simulink model "snap_adc5g_spec_rpi"  (R2019a)
settings: Solver=VariableStepDiscrete  StartTime=0.0  StopTime=10.0  RelTol=1e-3
undefined symbols (not defined in the file): pfb_coeff_gen_calc
libraries: xbsIndex_r4 x13965, casper_library_misc x80, casper_library_delays x43, xps_library x5, xbsReplacements_r4 x2, casper_library_communications x1
(part 94 of 152)

== system snap_adc5g_spec_rpi/fft_wideband_real/fft_direct/butterfly1_1/twiddle/coeff_gen/cosin ==
  theta : Inport
  misci : Inport  Port=2
  Constant : xbsIndex_r4/Constant  const=0  gui_display_data_type=Fixed-point  arith_type=Signed (2's comp)  n_bits=n_bits  bin_pt=bin_pt  preci_type=Single  exp_width=8  frac_width=24  explicit_period=off  period=1  equ=P=C  opselect=C  inp2=PCIN>>17  opr=+  inp1=P  carry=CIN  dbl_ovrd=off  block_type=constant
  Constant1 : xbsIndex_r4/Constant  const=0  gui_display_data_type=Fixed-point  arith_type=Signed (2's comp)  n_bits=n_bits  bin_pt=bin_pt  preci_type=Single  exp_width=8  frac_width=24  explicit_period=off  period=1  equ=P=C  opselect=C  inp2=PCIN>>17  opr=+  inp1=P  carry=CIN  dbl_ovrd=off  block_type=constant
  Constant2 : xbsIndex_r4/Constant  const=0  gui_display_data_type=Fixed-point  arith_type=Boolean  n_bits=n_bits  bin_pt=bin_pt  preci_type=Single  exp_width=8  frac_width=24  explicit_period=off  period=1  equ=P=C  opselect=C  inp2=PCIN>>17  opr=+  inp1=P  carry=CIN  dbl_ovrd=off  block_type=constant
  Constant3 : xbsIndex_r4/Constant  const=0  gui_display_data_type=Fixed-point  arith_type=Boolean  n_bits=n_bits  bin_pt=bin_pt  preci_type=Single  exp_width=8  frac_width=24  explicit_period=off  period=1  equ=P=C  opselect=C  inp2=PCIN>>17  opr=+  inp1=P  carry=CIN  dbl_ovrd=off  block_type=constant
  Constant4 : xbsIndex_r4/Constant  const=0  gui_display_data_type=Fixed-point  arith_type=Unsigned  n_bits=1  bin_pt=0  preci_type=Single  exp_width=8  frac_width=24  explicit_period=on  period=1  equ=P=C  opselect=C  inp2=PCIN>>17  opr=+  inp1=P  carry=CIN  dbl_ovrd=off  block_type=constant
  Constant5 : xbsIndex_r4/Constant  const=0  gui_display_data_type=Fixed-point  arith_type=Unsigned  n_bits=1  bin_pt=0  preci_type=Single  exp_width=8  frac_width=24  explicit_period=on  period=1  equ=P=C  opselect=C  inp2=PCIN>>17  opr=+  inp1=P  carry=CIN  dbl_ovrd=off  block_type=constant
  Delay : xbsIndex_r4/Delay  rst=off  infoeditControl=Selection of Reset will increase slice count due to use of real FFs and instead of SRLs  en=off  latency=bram_latency  reg_retiming=on  dbl_ovrd=off  block_type=delay
  Delay10 : xbsIndex_r4/Delay  rst=off  infoeditControl=Selection of Reset will increase slice count due to use of real FFs and instead of SRLs  en=off  latency=bram_latency  reg_retiming=on  dbl_ovrd=off  block_type=delay
  Delay8 : xbsIndex_r4/Delay  rst=off  infoeditControl=Selection of Reset will increase slice count due to use of real FFs and instead of SRLs  en=off  latency=bram_latency  reg_retiming=on  dbl_ovrd=off  block_type=delay
  Terminator : Terminator
  Terminator1 : Terminator
  add_convert0 : Subsystem
  add_convert1 : Subsystem
  assert : xbsIndex_r4/Assert  assert_type=on  type_source=Explicitly  gui_display_data_type=Fixed-point  arith_type=Unsigned  n_bits=11  bin_pt=0  preci_type=Single  exp_width=8  frac_width=24  assert_rate=off  rate_source=Explicitly  period=1  output_port=on  block_type=assert
  invert0 : Subsystem  mask{n_bits=n_bits, bin_pt=bin_pt, neg_latency=neg_latency, mux_latency=mux_latency}
      mask prompts: n_bits "bit width"; bin_pt "binary point"; neg_latency "negate latency"; mux_latency "mux latency"
  invert1 : Subsystem  mask{n_bits=n_bits, bin_pt=bin_pt, neg_latency=neg_latency, mux_latency=mux_latency}
      mask prompts: n_bits "bit width"; bin_pt "binary point"; neg_latency "negate latency"; mux_latency "mux latency"
  lookup : xbsIndex_r4/Dual Port RAM  depth=2^(11)  initVector=sin((0*(2*pi))+(2*pi)/(2^13)*(0:(2^11)-1))  distributed_mem=Block RAM  init_a=0  init_b=0  rst_a=off  rst_b=off  en_a=off  en_b=off  latency=bram_latency  write_mode_A=Read After Write  write_mode_B=Read After Write  optimize=Area  dbl_ovrd=off  block_type=dpram
  -sin : Outport
  -cos : Outport  Port=2
  misco : Outport  Port=3
  wires:
  theta/1 -> assert/1
  assert/1 -> add_convert0/1(theta), add_convert1/1(theta)
  Constant4/1 -> add_convert0/2(misci)
  add_convert0/3(misco) -> Terminator/1
  misci/1 -> add_convert1/2(misci)
  add_convert1/3(misco) -> Delay/1
  add_convert0/2(add) -> lookup/1
  add_convert1/2(add) -> lookup/4
  Constant/1 -> lookup/2
  Constant2/1 -> lookup/3
  Constant1/1 -> lookup/5
  Constant3/1 -> lookup/6
  add_convert1/1(negate) -> Delay8/1
  add_convert0/1(negate) -> Delay10/1
  Delay10/1 -> invert0/1(negate)
  Constant5/1 -> invert0/3(misci)
  lookup/1 -> invert0/2(in)
  Delay8/1 -> invert1/1(negate)
  lookup/2 -> invert1/2(in)
  invert0/2(misco) -> Terminator1/1
  Delay/1 -> invert1/3(misci)
  invert0/1(out) -> -sin/1
  invert1/1(out) -> -cos/1
  invert1/2(misco) -> misco/1

== system snap_adc5g_spec_rpi/fft_wideband_real/fft_unscrambler/reorder/buf0/rep_addr/bussify ==
  in1 : Inport
  in2 : Inport  Port=2
  in3 : Inport  Port=3
  in4 : Inport  Port=4
  in5 : Inport  Port=5
  in6 : Inport  Port=6
  in7 : Inport  Port=7
  in8 : Inport  Port=8
  concatenate : xbsIndex_r4/Concat  num_inputs=8  dbl_ovrd=off  block_type=concat
  reinterpret{1..8} (8 alike) : xbsIndex_r4/Reinterpret  force_arith_type=on  arith_type=Unsigned  force_bin_pt=on  bin_pt=0  block_type=reinterpret
      reinterpret1 settings: infoedit="Changes signal type without altering the binary representation.   You can changed the signal between signed and unsigned, and relocate the binary point.<br><br>Hardware notes: In hardware this block costs nothing.<br><br>Example:  Suppose the input is 6 bits wide, signed, with 2 fractional bits, and the output is forced to unsigned with 0 fractional bits.  Then an input of -2.0 (1110.00 in binary 2's complement) becomes an output of 56 (111000 in binary)."
      reinterpret2 settings: infoedit="Changes signal type without altering the binary representation.   You can changed the signal between signed and unsigned, and relocate the binary point.<br><br>Hardware notes: In hardware this block costs nothing.<br><br>Example:  Suppose the input is 6 bits wide, signed, with 2 fractional bits, and the output is forced to unsigned with 0 fractional bits.  Then an input of -2.0 (1110.00 in binary 2's complement) becomes an output of 56 (111000 in binary)."
  bus_out : Outport
  wires:
  concatenate/1 -> bus_out/1
  in1/1 -> reinterpret1/1
  reinterpret1/1 -> concatenate/1
  in2/1 -> reinterpret2/1
  reinterpret2/1 -> concatenate/2
  in3/1 -> reinterpret3/1
  reinterpret3/1 -> concatenate/3
  in4/1 -> reinterpret4/1
  reinterpret4/1 -> concatenate/4
  in5/1 -> reinterpret5/1
  reinterpret5/1 -> concatenate/5
  in6/1 -> reinterpret6/1
  reinterpret6/1 -> concatenate/6
  in7/1 -> reinterpret7/1
  reinterpret7/1 -> concatenate/7
  in8/1 -> reinterpret8/1
  reinterpret8/1 -> concatenate/8

== system snap_adc5g_spec_rpi/fft_wideband_real/fft_unscrambler/reorder/buf0/rep_we/bussify ==
  in1 : Inport
  in2 : Inport  Port=2
  in3 : Inport  Port=3
  in4 : Inport  Port=4
  in5 : Inport  Port=5
  in6 : Inport  Port=6
  in7 : Inport  Port=7
  in8 : Inport  Port=8
  concatenate : xbsIndex_r4/Concat  num_inputs=8  dbl_ovrd=off  block_type=concat
  reinterpret{1..8} (8 alike) : xbsIndex_r4/Reinterpret  force_arith_type=on  arith_type=Unsigned  force_bin_pt=on  bin_pt=0  block_type=reinterpret
      reinterpret1 settings: infoedit="Changes signal type without altering the binary representation.   You can changed the signal between signed and unsigned, and relocate the binary point.<br><br>Hardware notes: In hardware this block costs nothing.<br><br>Example:  Suppose the input is 6 bits wide, signed, with 2 fractional bits, and the output is forced to unsigned with 0 fractional bits.  Then an input of -2.0 (1110.00 in binary 2's complement) becomes an output of 56 (111000 in binary)."
      reinterpret2 settings: infoedit="Changes signal type without altering the binary representation.   You can changed the signal between signed and unsigned, and relocate the binary point.<br><br>Hardware notes: In hardware this block costs nothing.<br><br>Example:  Suppose the input is 6 bits wide, signed, with 2 fractional bits, and the output is forced to unsigned with 0 fractional bits.  Then an input of -2.0 (1110.00 in binary 2's complement) becomes an output of 56 (111000 in binary)."
  bus_out : Outport
  wires:
  concatenate/1 -> bus_out/1
  in1/1 -> reinterpret1/1
  reinterpret1/1 -> concatenate/1
  in2/1 -> reinterpret2/1
  reinterpret2/1 -> concatenate/2
  in3/1 -> reinterpret3/1
  reinterpret3/1 -> concatenate/3
  in4/1 -> reinterpret4/1
  reinterpret4/1 -> concatenate/4
  in5/1 -> reinterpret5/1
  reinterpret5/1 -> concatenate/5
  in6/1 -> reinterpret6/1
  reinterpret6/1 -> concatenate/6
  in7/1 -> reinterpret7/1
  reinterpret7/1 -> concatenate/7
  in8/1 -> reinterpret8/1
  reinterpret8/1 -> concatenate/8

== system snap_adc5g_spec_rpi/fft_wideband_real/fft_unscrambler/reorder/buf1/rep_addr/bussify ==
  in1 : Inport
  in2 : Inport  Port=2
  in3 : Inport  Port=3
  in4 : Inport  Port=4
  in5 : Inport  Port=5
  in6 : Inport  Port=6
  in7 : Inport  Port=7
  in8 : Inport  Port=8
  concatenate : xbsIndex_r4/Concat  num_inputs=8  dbl_ovrd=off  block_type=concat
  reinterpret{1..8} (8 alike) : xbsIndex_r4/Reinterpret  force_arith_type=on  arith_type=Unsigned  force_bin_pt=on  bin_pt=0  block_type=reinterpret
      reinterpret1 settings: infoedit="Changes signal type without altering the binary representation.   You can changed the signal between signed and unsigned, and relocate the binary point.<br><br>Hardware notes: In hardware this block costs nothing.<br><br>Example:  Suppose the input is 6 bits wide, signed, with 2 fractional bits, and the output is forced to unsigned with 0 fractional bits.  Then an input of -2.0 (1110.00 in binary 2's complement) becomes an output of 56 (111000 in binary)."
      reinterpret2 settings: infoedit="Changes signal type without altering the binary representation.   You can changed the signal between signed and unsigned, and relocate the binary point.<br><br>Hardware notes: In hardware this block costs nothing.<br><br>Example:  Suppose the input is 6 bits wide, signed, with 2 fractional bits, and the output is forced to unsigned with 0 fractional bits.  Then an input of -2.0 (1110.00 in binary 2's complement) becomes an output of 56 (111000 in binary)."
  bus_out : Outport
  wires:
  concatenate/1 -> bus_out/1
  in1/1 -> reinterpret1/1
  reinterpret1/1 -> concatenate/1
  in2/1 -> reinterpret2/1
  reinterpret2/1 -> concatenate/2
  in3/1 -> reinterpret3/1
  reinterpret3/1 -> concatenate/3
  in4/1 -> reinterpret4/1
  reinterpret4/1 -> concatenate/4
  in5/1 -> reinterpret5/1
  reinterpret5/1 -> concatenate/5
  in6/1 -> reinterpret6/1
  reinterpret6/1 -> concatenate/6
  in7/1 -> reinterpret7/1
  reinterpret7/1 -> concatenate/7
  in8/1 -> reinterpret8/1
  reinterpret8/1 -> concatenate/8

== system snap_adc5g_spec_rpi/fft_wideband_real/fft_unscrambler/reorder/buf1/rep_we/bussify ==
  in1 : Inport
  in2 : Inport  Port=2
  in3 : Inport  Port=3
  in4 : Inport  Port=4
  in5 : Inport  Port=5
  in6 : Inport  Port=6
  in7 : Inport  Port=7
  in8 : Inport  Port=8
  concatenate : xbsIndex_r4/Concat  num_inputs=8  dbl_ovrd=off  block_type=concat
  reinterpret{1..8} (8 alike) : xbsIndex_r4/Reinterpret  force_arith_type=on  arith_type=Unsigned  force_bin_pt=on  bin_pt=0  block_type=reinterpret
      reinterpret1 settings: infoedit="Changes signal type without altering the binary representation.   You can changed the signal between signed and unsigned, and relocate the binary point.<br><br>Hardware notes: In hardware this block costs nothing.<br><br>Example:  Suppose the input is 6 bits wide, signed, with 2 fractional bits, and the output is forced to unsigned with 0 fractional bits.  Then an input of -2.0 (1110.00 in binary 2's complement) becomes an output of 56 (111000 in binary)."
      reinterpret2 settings: infoedit="Changes signal type without altering the binary representation.   You can changed the signal between signed and unsigned, and relocate the binary point.<br><br>Hardware notes: In hardware this block costs nothing.<br><br>Example:  Suppose the input is 6 bits wide, signed, with 2 fractional bits, and the output is forced to unsigned with 0 fractional bits.  Then an input of -2.0 (1110.00 in binary 2's complement) becomes an output of 56 (111000 in binary)."
  bus_out : Outport
  wires:
  concatenate/1 -> bus_out/1
  in1/1 -> reinterpret1/1
  reinterpret1/1 -> concatenate/1
  in2/1 -> reinterpret2/1
  reinterpret2/1 -> concatenate/2
  in3/1 -> reinterpret3/1
  reinterpret3/1 -> concatenate/3
  in4/1 -> reinterpret4/1
  reinterpret4/1 -> concatenate/4
  in5/1 -> reinterpret5/1
  reinterpret5/1 -> concatenate/5
  in6/1 -> reinterpret6/1
  reinterpret6/1 -> concatenate/6
  in7/1 -> reinterpret7/1
  reinterpret7/1 -> concatenate/7
  in8/1 -> reinterpret8/1
  reinterpret8/1 -> concatenate/8

== system snap_adc5g_spec_rpi/fft_wideband_real/fft_unscrambler/reorder/current_map/rep_addra0/bussify ==
  in1 : Inport
  reinterpret1 : xbsIndex_r4/Reinterpret  force_arith_type=on  arith_type=Unsigned  force_bin_pt=on  bin_pt=0  block_type=reinterpret
      settings: infoedit="Changes signal type without altering the binary representation.   You can changed the signal between signed and unsigned, and relocate the binary point.<br><br>Hardware notes: In hardware this block costs nothing.<br><br>Example:  Suppose the input is 6 bits wide, signed, with 2 fractional bits, and the output is forced to unsigned with 0 fractional bits.  Then an input of -2.0 (1110.00 in binary 2's complement) becomes an output of 56 (111000 in binary)."
  bus_out : Outport
  wires:
  in1/1 -> reinterpret1/1
  reinterpret1/1 -> bus_out/1

== system snap_adc5g_spec_rpi/fft_wideband_real/fft_unscrambler/reorder/current_map/rep_addrb0/bussify ==
  in1 : Inport
  reinterpret1 : xbsIndex_r4/Reinterpret  force_arith_type=on  arith_type=Unsigned  force_bin_pt=on  bin_pt=0  block_type=reinterpret
      settings: infoedit="Changes signal type without altering the binary representation.   You can changed the signal between signed and unsigned, and relocate the binary point.<br><br>Hardware notes: In hardware this block costs nothing.<br><br>Example:  Suppose the input is 6 bits wide, signed, with 2 fractional bits, and the output is forced to unsigned with 0 fractional bits.  Then an input of -2.0 (1110.00 in binary 2's complement) becomes an output of 56 (111000 in binary)."
  bus_out : Outport
  wires:
  in1/1 -> reinterpret1/1
  reinterpret1/1 -> bus_out/1

== system snap_adc5g_spec_rpi/fft_wideband_real/fft_unscrambler/reorder/current_map/rep_wea0/bussify ==
  in1 : Inport
  reinterpret1 : xbsIndex_r4/Reinterpret  force_arith_type=on  arith_type=Unsigned  force_bin_pt=on  bin_pt=0  block_type=reinterpret
      settings: infoedit="Changes signal type without altering the binary representation.   You can changed the signal between signed and unsigned, and relocate the binary point.<br><br>Hardware notes: In hardware this block costs nothing.<br><br>Example:  Suppose the input is 6 bits wide, signed, with 2 fractional bits, and the output is forced to unsigned with 0 fractional bits.  Then an input of -2.0 (1110.00 in binary 2's complement) becomes an output of 56 (111000 in binary)."
  bus_out : Outport
  wires:
  in1/1 -> reinterpret1/1
  reinterpret1/1 -> bus_out/1

== system snap_adc5g_spec_rpi/fft_wideband_real/fft_unscrambler/reorder/current_map/rep_web0/bussify ==
  in1 : Inport
  reinterpret1 : xbsIndex_r4/Reinterpret  force_arith_type=on  arith_type=Unsigned  force_bin_pt=on  bin_pt=0  block_type=reinterpret
      settings: infoedit="Changes signal type without altering the binary representation.   You can changed the signal between signed and unsigned, and relocate the binary point.<br><br>Hardware notes: In hardware this block costs nothing.<br><br>Example:  Suppose the input is 6 bits wide, signed, with 2 fractional bits, and the output is forced to unsigned with 0 fractional bits.  Then an input of -2.0 (1110.00 in binary 2's complement) becomes an output of 56 (111000 in binary)."
  bus_out : Outport
  wires:
  in1/1 -> reinterpret1/1
  reinterpret1/1 -> bus_out/1

== system snap_adc5g_spec_rpi/tge/core/txs/ss/add_gen/edge_detect ==
  in : Inport
  Delay : xbsIndex_r4/Delay  rst=off  infoeditControl=Selection of Reset will increase slice count due to use of real FFs and instead of SRLs  en=off  latency=1  reg_retiming=off  dbl_ovrd=off  block_type=delay
      settings: xl_area=[0, 0, 0, 0, 0, 0, 0]
  Inverter : xbsIndex_r4/Inverter  en=off  latency=0  dbl_ovrd=off  block_type=inv
      settings: xl_area=[0, 0, 0, 0, 0, 0, 0]
  edge_op : xbsIndex_r4/Logical  logical_function=XNOR  inputs=2  en=off  latency=0  precision=Full  arith_type=Unsigned  n_bits=8  bin_pt=2  align_bp=on  dbl_ovrd=off  block_type=logical
      settings: xl_area=[0, 0, 0, 0, 0, 0, 0]
  out : Outport
  wires:
  Delay/1 -> edge_op/2
  in/1 -> Delay/1, Inverter/1
  edge_op/1 -> out/1
  Inverter/1 -> edge_op/1

== system snap_adc5g_spec_rpi/tge/core/txs/ss/add_gen/edge_detect1 ==
  in : Inport
  Delay : xbsIndex_r4/Delay  rst=off  infoeditControl=Selection of Reset will increase slice count due to use of real FFs and instead of SRLs  en=off  latency=1  reg_retiming=off  dbl_ovrd=off  block_type=delay
      settings: xl_area=[0, 0, 0, 0, 0, 0, 0]
  Inverter : xbsIndex_r4/Inverter  en=off  latency=0  dbl_ovrd=off  block_type=inv
      settings: xl_area=[0, 0, 0, 0, 0, 0, 0]
  edge_op : xbsIndex_r4/Logical  logical_function=XNOR  inputs=2  en=off  latency=0  precision=Full  arith_type=Unsigned  n_bits=8  bin_pt=2  align_bp=on  dbl_ovrd=off  block_type=logical
      settings: xl_area=[0, 0, 0, 0, 0, 0, 0]
  out : Outport
  wires:
  Inverter/1 -> edge_op/1
  edge_op/1 -> out/1
  in/1 -> Inverter/1, Delay/1
  Delay/1 -> edge_op/2

== system snap_adc5g_spec_rpi/tge/core/txs/ss/basic_ctrl/dram_munge ==
  note: 1st output same time
      | as last input
  note: Choose DRAM data
      | or standard. Constant input
      | to muxes should ensure
      | other path optimised
      | away
  note: Buffer 4 input words when using DRAM
      | then combine and output the first two,
      | then second. Ensures that a full burst
      | goes through every time so that status
      | register records number of bytes fully in
      | DRAM
  vin : Inport
  din : Inport  Port=2
  we : Inport  Port=3
  init : Inport  Port=4
  Concat : xbsIndex_r4/Concat  num_inputs=4  dbl_ovrd=off  block_type=concat
  Concat1 : xbsIndex_r4/Concat  num_inputs=4  dbl_ovrd=off  block_type=concat
  Constant : xbsIndex_r4/Constant  const=0  gui_display_data_type=Fixed-point  arith_type=Unsigned  n_bits=8  bin_pt=0  preci_type=Single  exp_width=8  frac_width=24  explicit_period=on  period=1  equ=P=C  opselect=C  inp2=PCIN>>17  opr=+  inp1=P  carry=CIN  dbl_ovrd=off  block_type=constant
      settings: block_version=11.4
  Delay : xbsIndex_r4/Delay  rst=off  infoeditControl=Selection of Reset will increase slice count due to use of real FFs and instead of SRLs  en=off  latency=1  reg_retiming=off  dbl_ovrd=off  block_type=delay
      settings: block_version=11.4
  Delay1 : xbsIndex_r4/Delay  rst=off  infoeditControl=Selection of Reset will increase slice count due to use of real FFs and instead of SRLs  en=off  latency=1  reg_retiming=off  dbl_ovrd=off  block_type=delay
      settings: block_version=11.4
  Logical : xbsIndex_r4/Logical  logical_function=AND  inputs=2  en=off  latency=1  precision=Full  arith_type=Unsigned  n_bits=16  bin_pt=0  align_bp=on  dbl_ovrd=off  block_type=logical
      settings: block_version=11.4
  Logical1 : xbsIndex_r4/Logical  logical_function=OR  inputs=2  en=off  latency=0  precision=Full  arith_type=Unsigned  n_bits=16  bin_pt=0  align_bp=on  dbl_ovrd=off  block_type=logical
      settings: block_version=11.4
  Logical2 : xbsIndex_r4/Logical  logical_function=AND  inputs=2  en=off  latency=0  precision=Full  arith_type=Unsigned  n_bits=16  bin_pt=0  align_bp=on  dbl_ovrd=off  block_type=logical
      settings: block_version=11.4
  Mux1 : xbsIndex_r4/Mux  inputs=2  en=off  latency=1  precision=Full  arith_type=Unsigned  n_bits=16  bin_pt=14  quantization=Truncate  overflow=Wrap  dbl_ovrd=off  block_type=mux
      settings: block_version=11.4
  Register{,1..3,5} (5 alike) : xbsIndex_r4/Register  init=0  rst=off  en=on  dbl_ovrd=off  block_type=register
      settings: block_version=11.4
  Register4 : xbsIndex_r4/Register  init=0  rst=on  en=on  dbl_ovrd=off  block_type=register
      settings: block_version=11.4
  Relational{,1..3} (4 alike) : xbsIndex_r4/Relational  mode=a=b  op_type=Bool  en=off  latency=0  dbl_ovrd=off  block_type=relational
  con0 : xbsIndex_r4/Constant  const=0  gui_display_data_type=Fixed-point  arith_type=Unsigned  n_bits=2  bin_pt=0  preci_type=Single  exp_width=8  frac_width=24  explicit_period=on  period=1  equ=P=C  opselect=C  inp2=PCIN>>17  opr=+  inp1=P  carry=CIN  dbl_ovrd=off  block_type=constant
      settings: block_version=11.4
  con1 : xbsIndex_r4/Constant  const=1  gui_display_data_type=Fixed-point  arith_type=Unsigned  n_bits=2  bin_pt=0  preci_type=Single  exp_width=8  frac_width=24  explicit_period=on  period=1  equ=P=C  opselect=C  inp2=PCIN>>17  opr=+  inp1=P  carry=CIN  dbl_ovrd=off  block_type=constant
      settings: block_version=11.4
  con2 : xbsIndex_r4/Constant  const=2  gui_display_data_type=Fixed-point  arith_type=Unsigned  n_bits=2  bin_pt=0  preci_type=Single  exp_width=8  frac_width=24  explicit_period=on  period=1  equ=P=C  opselect=C  inp2=PCIN>>17  opr=+  inp1=P  carry=CIN  dbl_ovrd=off  block_type=constant
      settings: block_version=11.4
  con3 : xbsIndex_r4/Constant  const=3  gui_display_data_type=Fixed-point  arith_type=Unsigned  n_bits=2  bin_pt=0  preci_type=Single  exp_width=8  frac_width=24  explicit_period=on  period=1  equ=P=C  opselect=C  inp2=PCIN>>17  opr=+  inp1=P  carry=CIN  dbl_ovrd=off  block_type=constant
      settings: block_version=11.4
  data_choice : xbsIndex_r4/Mux  inputs=2  en=off  latency=0  precision=User Defined  arith_type=Unsigned  n_bits=128  bin_pt=0  quantization=Truncate  overflow=Wrap  dbl_ovrd=off  block_type=mux
      settings: block_version=11.4
  dout_count : xbsIndex_r4/Counter  cnt_type=Free Running  cnt_to=Inf  operation=Up  start_count=0  cnt_by_val=1  arith_type=Unsigned  n_bits=1  bin_pt=0  load_pin=off  rst=on  en=on  explicit_period=on  period=1  use_behavioral_HDL=off  implementation=Fabric  dbl_ovrd=off  block_type=counter
      settings: block_version=11.4
  dram : xbsIndex_r4/Constant  const=0  gui_display_data_type=Fixed-point  arith_type=Boolean  n_bits=16  bin_pt=14  preci_type=Single  exp_width=8  frac_width=24  explicit_period=on  period=1  equ=P=C  opselect=C  inp2=PCIN>>17  opr=+  inp1=P  carry=CIN  dbl_ovrd=off  block_type=constant
      settings: block_version=11.4
  input_count : xbsIndex_r4/Counter  cnt_type=Free Running  cnt_to=Inf  operation=Up  start_count=0  cnt_by_val=1  arith_type=Unsigned  n_bits=2  bin_pt=0  load_pin=off  rst=on  en=on  explicit_period=on  period=1  use_behavioral_HDL=off  implementation=Fabric  dbl_ovrd=off  block_type=counter
      settings: block_version=11.4
  vout_choice : xbsIndex_r4/Mux  inputs=2  en=off  latency=0  precision=Full  arith_type=Unsigned  n_bits=16  bin_pt=14  quantization=Truncate  overflow=Wrap  dbl_ovrd=off  block_type=mux
      settings: block_version=11.4
  we_choice : xbsIndex_r4/Mux  inputs=2  en=off  latency=0  precision=Full  arith_type=Unsigned  n_bits=16  bin_pt=14  quantization=Truncate  overflow=Wrap  dbl_ovrd=off  block_type=mux
      settings: block_version=11.4
  vout : Outport
  dout : Outport  Port=2
  we_o : Outport  Port=3
  wires:
  Register3/1 -> Concat1/4
  Register2/1 -> Concat1/2
  Constant/1 -> Concat1/3, Concat1/1, Concat/3, Concat/1
  Register1/1 -> Concat/4
  Register/1 -> Concat/2
  [vin] -> vout_choice/2
  Register5/1 -> vout_choice/3
  vout_choice/1 -> vout/1
  Logical2/1 -> Register5/2
  [we] -> Logical2/2, Register4/2
  vin/1 -> [vin], Register5/1
  Register4/1 -> Logical2/1
  [init] -> Register4/3, Register4/1
  dram/1 -> vout_choice/1, we_choice/1, data_choice/1
  [din] -> data_choice/2
  Mux1/1 -> data_choice/3
  [we] -> we_choice/2
  Delay1/1 -> we_choice/3
  we_choice/1 -> we_o/1
  dout_count/1 -> Mux1/1
  [init] -> dout_count/1
  Logical1/1 -> Delay1/1, dout_count/2
  Concat1/1 -> Mux1/3
  Concat/1 -> Mux1/2
  Delay/1 -> Logical1/2
  Logical/1 -> Logical1/1, Delay/1
  Relational3/1 -> Logical/1, Register3/2
  Relational2/1 -> Register2/2
  Relational1/1 -> Register1/2
  Relational/1 -> Register/2
  con3/1 -> Relational3/2
  con2/1 -> Relational2/2
  con1/1 -> Relational1/2
  con0/1 -> Relational/2
  input_count/1 -> Relational3/1, Relational2/1, Relational1/1, Relational/1
  din/1 -> [din], Register3/1, Register2/1, Register1/1, Register/1
  we/1 -> [we], Logical/2, input_count/2
  init/1 -> [init], input_count/1
  data_choice/1 -> dout/1

== system snap_adc5g_spec_rpi/tge/core/txs/ss/bram/calc_add ==
  note: If reading/writing words
      | smaller than 32 bits,
      | change address so
      | that addressing is
      | big endian instead of
      | little, otherwise
      | pass through
  note: Use behavioural HDL
      | so that gets optimised
      | to minimum logic
  in : Inport
  add_sub : xbsIndex_r4/AddSub  mode=Subtraction  use_carryin=off  use_carryout=off  en=off  latency=0  precision=User Defined  arith_type=Unsigned  n_bits=max(1, log2(32/data_width))  bin_pt=0  quantization=Truncate  overflow=Wrap  use_behavioral_HDL=on  hw_selection=Fabric  pipelined=off  dbl_ovrd=off  block_type=addsub
  concat : xbsIndex_r4/Concat  num_inputs=2  dbl_ovrd=off  block_type=concat
  const : xbsIndex_r4/Constant  const=max(0, 32/data_width-1)  gui_display_data_type=Fixed-point  arith_type=Unsigned  n_bits=max(1, log2(32/data_width))  bin_pt=0  preci_type=Single  exp_width=8  frac_width=24  explicit_period=on  period=sample_rate  equ=P=C  opselect=C  inp2=PCIN>>17  opr=+  inp1=P  carry=CIN  dbl_ovrd=off  block_type=constant
      settings: block_version=11.4
  convert_addr : xbsIndex_r4/Convert  gui_display_data_type=Fixed-point  arith_type=Unsigned  n_bits=addr_width  bin_pt=0  float_type=Single  exp_bits=8  fraction_bits=24  quantization=Truncate  overflow=Wrap  en=off  latency=0  pipeline=off  dbl_ovrd=off  block_type=convert
      settings: xl_area=[0, 0, 0, 0, 0, 0, 0]
  lsw : xbsIndex_r4/Slice  nbits=max(1, log2(32/data_width))  boolean_output=off  mode=Lower Bit Location + Width  bit1=0  base1=MSB of Input  bit0=0  base0=LSB of Input  dbl_ovrd=off  block_type=slice
  manipulate : xbsIndex_r4/Constant  const=min(1, floor(32/data_width) - 1)  gui_display_data_type=Fixed-point  arith_type=Unsigned  n_bits=1  bin_pt=0  preci_type=Single  exp_width=8  frac_width=24  explicit_period=on  period=sample_rate  equ=P=C  opselect=C  inp2=PCIN>>17  opr=+  inp1=P  carry=CIN  dbl_ovrd=off  block_type=constant
      settings: block_version=11.4
  msw : xbsIndex_r4/Slice  nbits=addr_width - max(1, log2(32/data_width))  boolean_output=off  mode=Upper Bit Location + Width  bit1=0  base1=MSB of Input  bit0=0  base0=LSB of Input  dbl_ovrd=off  block_type=slice
  mux : xbsIndex_r4/Mux  inputs=2  en=off  latency=0  precision=Full  arith_type=Unsigned  n_bits=16  bin_pt=14  quantization=Truncate  overflow=Wrap  dbl_ovrd=off  block_type=mux
      settings: block_version=11.4
  out : Outport
  wires:
  in/1 -> convert_addr/1
  add_sub/1 -> concat/2
  msw/1 -> concat/1
  concat/1 -> mux/3
  manipulate/1 -> mux/1
  mux/1 -> out/1
  lsw/1 -> add_sub/2
  const/1 -> add_sub/1
  convert_addr/1 -> lsw/1, msw/1, mux/2

== system snap_adc5g_spec_rpi/tge/core/txs/ss/bram/munge_in ==
  din : Inport
  join : Subsystem  AncestorBlock=casper_library_flow_control/bus_create  mask(bus_create){inputNum=4}
      mask prompts: inputNum "Number of inputs:"
      mask init:
      | bus_create_init(gcb,...
      |     'inputNum', inputNum);
  reinterpret : xbsIndex_r4/Reinterpret  force_arith_type=on  arith_type=Unsigned  force_bin_pt=on  bin_pt=0  block_type=reinterpret
  reinterpret_out : xbsIndex_r4/Reinterpret  force_arith_type=on  arith_type=Unsigned  force_bin_pt=on  bin_pt=0  block_type=reinterpret
  split : Subsystem  AncestorBlock=casper_library_flow_control/bus_expand  mask(bus_expand){mode=divisions of arbitrary size, outputNum=1, outputWidth=[32 32 32 32], outputBinaryPt=[0 0 0 0], outputArithmeticType=[0 0 0 0], show_format=off, outputToWorkspace=off, variablePrefix=out, outputToModelAsWell=on}
      mask prompts: outputNum "Number of outputs:"; outputWidth "Output width [msb ... lsb]:"; outputBinaryPt "Output binary point position [msb ... lsb]:"; outputArithmeticType "Output arithmetic type (ufix=0, fix=1, bool=2) [msb ... lsb]:"; show_format "Print format string?"; outputToWorkspace "Output to workspace?"; variablePrefix "Variable name prefix:"; outputToModelAsWell "Output to model as well?"
      mask help:
      | Expands a 'bus' made using a bus_create or Xilinx
      | concat block.
      | The input will be divided into the specified number
      | of outputs with the specified arithmetic types.
      | Divisions are made from most significant bit.
      mask init: same as snap_adc5g_spec_rpi/ss_adc/ctrl_split
      settings: AttributesFormatString=4 outputs
      mask TypeOptions mode: divisions of equal size | divisions of arbitrary size
      mask Callback mode: bus_expand_callback();
      mask Callback outputWidth: bus_expand_callback();
      mask Callback outputToWorkspace: bus_expand_callback();
  dout : Outport
  wires:
  reinterpret_out/1 -> dout/1
  din/1 -> reinterpret/1
  reinterpret/1 -> split/1(bus_in)
  join/1(bus_out) -> reinterpret_out/1
  split/4(lsb_out1) -> join/1(in1)
  split/3(out2) -> join/2(in2)
  split/2(out3) -> join/3(in3)
  split/1(msb_out4) -> join/4(in4)

== system snap_adc5g_spec_rpi/tge/core/txs/ss/bram/munge_out ==
  din : Inport
  join : Subsystem  AncestorBlock=casper_library_flow_control/bus_create  mask(bus_create){inputNum=4}
      mask prompts: inputNum "Number of inputs:"
      mask init:
      | bus_create_init(gcb,...
      |     'inputNum', inputNum);
  reinterpret : xbsIndex_r4/Reinterpret  force_arith_type=on  arith_type=Unsigned  force_bin_pt=on  bin_pt=0  block_type=reinterpret
  reinterpret_out : xbsIndex_r4/Reinterpret  force_arith_type=on  arith_type=Unsigned  force_bin_pt=on  bin_pt=0  block_type=reinterpret
  split : Subsystem  AncestorBlock=casper_library_flow_control/bus_expand  mask(bus_expand){mode=divisions of arbitrary size, outputNum=1, outputWidth=[32 32 32 32], outputBinaryPt=[0 0 0 0], outputArithmeticType=[0 0 0 0], show_format=off, outputToWorkspace=off, variablePrefix=out, outputToModelAsWell=on}
      mask prompts: outputNum "Number of outputs:"; outputWidth "Output width [msb ... lsb]:"; outputBinaryPt "Output binary point position [msb ... lsb]:"; outputArithmeticType "Output arithmetic type (ufix=0, fix=1, bool=2) [msb ... lsb]:"; show_format "Print format string?"; outputToWorkspace "Output to workspace?"; variablePrefix "Variable name prefix:"; outputToModelAsWell "Output to model as well?"
      mask help:
      | Expands a 'bus' made using a bus_create or Xilinx
      | concat block.
      | The input will be divided into the specified number
      | of outputs with the specified arithmetic types.
      | Divisions are made from most significant bit.
      mask init: same as snap_adc5g_spec_rpi/ss_adc/ctrl_split
      settings: AttributesFormatString=4 outputs
      mask TypeOptions mode: divisions of equal size | divisions of arbitrary size
      mask Callback mode: bus_expand_callback();
      mask Callback outputWidth: bus_expand_callback();
      mask Callback outputToWorkspace: bus_expand_callback();
  dout : Outport
  wires:
  reinterpret_out/1 -> dout/1
  din/1 -> reinterpret/1
  reinterpret/1 -> split/1(bus_in)
  join/1(bus_out) -> reinterpret_out/1
  split/4(lsb_out1) -> join/1(in1)
  split/3(out2) -> join/2(in2)
  split/2(out3) -> join/3(in3)
  split/1(msb_out4) -> join/4(in4)

== system snap_adc5g_spec_rpi/tge/core/txs/ss/bram/sim_mem ==
  addr : Inport
  data : Inport  Port=2
  we : Inport  Port=3
  Data Type Conversion : DataTypeConversion  OutDataTypeStr=single
  Data Type Conversion1 : DataTypeConversion  OutDataTypeStr=double
  Data Type Conversion2 : DataTypeConversion  OutDataTypeStr=boolean
  sfunc : M-S-Function  FunctionName=shared_bram_sim_sfunc  Parameters=depth_bits, latency, init_vals  mask{depth_bits=addr_width, latency=csp_latency, init_vals=init_vals}
      mask prompts: depth_bits "Depth (2^?):"; latency "Latency (>=1):"; init_vals "Initial values:"
      mask Callback latency:
      | latency = str2double(get_param(gcb, 'latency'));
      | if latency < 1
      |     errordlg('Cannot have latency less than one.');
      |     set_param(gcb, 'latency', '1');
      | end
  sim_addr : xbsIndex_r4/Gateway Out  inherit_from_input=off  hdl_port=off  rows=1  columns=1  UseAsDAC=off  DACChannel='1'  interface=None  automatic_assignment=on  address_offset=hex2dec('00')  intf_name=''  intf_description=''  timing_constraint=None  locs_specified=off  LOCs={}  io_standard={}  block_type=gatewayout
  sim_data : xbsIndex_r4/Gateway Out  inherit_from_input=off  hdl_port=off  rows=1  columns=1  UseAsDAC=off  DACChannel='1'  interface=None  automatic_assignment=on  address_offset=hex2dec('00')  intf_name=''  intf_description=''  timing_constraint=None  locs_specified=off  LOCs={}  io_standard={}  block_type=gatewayout
  sim_we : xbsIndex_r4/Gateway Out  inherit_from_input=off  hdl_port=off  rows=1  columns=1  UseAsDAC=off  DACChannel='1'  interface=None  automatic_assignment=on  address_offset=hex2dec('00')  intf_name=''  intf_description=''  timing_constraint=None  locs_specified=off  LOCs={}  io_standard={}  block_type=gatewayout
  data_out : Outport
  wires:
  addr/1 -> sim_addr/1
  data/1 -> sim_data/1
  we/1 -> sim_we/1
  sim_addr/1 -> Data Type Conversion/1
  sim_data/1 -> Data Type Conversion1/1
  sim_we/1 -> Data Type Conversion2/1
  Data Type Conversion/1 -> sfunc/1  "addr"
  Data Type Conversion1/1 -> sfunc/2  "data_in"
  Data Type Conversion2/1 -> sfunc/3  "we"
  sfunc/1 -> data_out/1  "output"

== system snap_adc5g_spec_rpi/fft_wideband_real/fft_biplex_real_4x/bi_real_unscr_4x/mirror_spectrum/complex_conj0/imag_negate/bussify ==
  in1 : Inport
  in2 : Inport  Port=2
  concatenate : xbsIndex_r4/Concat  num_inputs=2  dbl_ovrd=off  block_type=concat
  reinterpret1 : xbsIndex_r4/Reinterpret  force_arith_type=on  arith_type=Unsigned  force_bin_pt=on  bin_pt=0  block_type=reinterpret
      settings: infoedit="Changes signal type without altering the binary representation.   You can changed the signal between signed and unsigned, and relocate the binary point.<br><br>Hardware notes: In hardware this block costs nothing.<br><br>Example:  Suppose the input is 6 bits wide, signed, with 2 fractional bits, and the output is forced to unsigned with 0 fractional bits.  Then an input of -2.0 (1110.00 in binary 2's complement) becomes an output of 56 (111000 in binary)."
  reinterpret2 : xbsIndex_r4/Reinterpret  force_arith_type=on  arith_type=Unsigned  force_bin_pt=on  bin_pt=0  block_type=reinterpret
      settings: infoedit="Changes signal type without altering the binary representation.   You can changed the signal between signed and unsigned, and relocate the binary point.<br><br>Hardware notes: In hardware this block costs nothing.<br><br>Example:  Suppose the input is 6 bits wide, signed, with 2 fractional bits, and the output is forced to unsigned with 0 fractional bits.  Then an input of -2.0 (1110.00 in binary 2's complement) becomes an output of 56 (111000 in binary)."
  bus_out : Outport
  wires:
  concatenate/1 -> bus_out/1
  in1/1 -> reinterpret1/1
  reinterpret1/1 -> concatenate/1
  in2/1 -> reinterpret2/1
  reinterpret2/1 -> concatenate/2

== system snap_adc5g_spec_rpi/fft_wideband_real/fft_biplex_real_4x/bi_real_unscr_4x/mirror_spectrum/complex_conj0/imag_negate/debus ==
  bus_in : Inport
  reinterpret1 : xbsIndex_r4/Reinterpret  force_arith_type=on  arith_type="Signed  (2's comp)"  force_bin_pt=on  bin_pt=17  block_type=reinterpret
  reinterpret2 : xbsIndex_r4/Reinterpret  force_arith_type=on  arith_type="Signed  (2's comp)"  force_bin_pt=on  bin_pt=17  block_type=reinterpret
  slice1 : xbsIndex_r4/Slice  nbits=18  boolean_output=off  mode=Upper Bit Location + Width  bit1=-18  base1=MSB of Input  bit0=0  base0=LSB of Input  dbl_ovrd=off  block_type=slice
  slice2 : xbsIndex_r4/Slice  nbits=18  boolean_output=off  mode=Upper Bit Location + Width  bit1=0  base1=MSB of Input  bit0=0  base0=LSB of Input  dbl_ovrd=off  block_type=slice
  msb_out2 : Outport
  lsb_out1 : Outport  Port=2
  wires:
  bus_in/1 -> slice2/1, slice1/1
  slice2/1 -> reinterpret2/1
  reinterpret2/1 -> msb_out2/1
  slice1/1 -> reinterpret1/1
  reinterpret1/1 -> lsb_out1/1

== system snap_adc5g_spec_rpi/fft_wideband_real/fft_biplex_real_4x/bi_real_unscr_4x/mirror_spectrum/complex_conj0/munge_in/join ==
  in1 : Inport
  in2 : Inport  Port=2
  in3 : Inport  Port=3
  in4 : Inport  Port=4
  concatenate : xbsIndex_r4/Concat  num_inputs=4  dbl_ovrd=off  block_type=concat
  reinterpret{1..4} (4 alike) : xbsIndex_r4/Reinterpret  force_arith_type=on  arith_type=Unsigned  force_bin_pt=on  bin_pt=0  block_type=reinterpret
      reinterpret1 settings: infoedit="Changes signal type without altering the binary representation.   You can changed the signal between signed and unsigned, and relocate the binary point.<br><br>Hardware notes: In hardware this block costs nothing.<br><br>Example:  Suppose the input is 6 bits wide, signed, with 2 fractional bits, and the output is forced to unsigned with 0 fractional bits.  Then an input of -2.0 (1110.00 in binary 2's complement) becomes an output of 56 (111000 in binary)."
      reinterpret2 settings: infoedit="Changes signal type without altering the binary representation.   You can changed the signal between signed and unsigned, and relocate the binary point.<br><br>Hardware notes: In hardware this block costs nothing.<br><br>Example:  Suppose the input is 6 bits wide, signed, with 2 fractional bits, and the output is forced to unsigned with 0 fractional bits.  Then an input of -2.0 (1110.00 in binary 2's complement) becomes an output of 56 (111000 in binary)."
  bus_out : Outport
  wires:
  concatenate/1 -> bus_out/1
  in1/1 -> reinterpret1/1
  reinterpret1/1 -> concatenate/1
  in2/1 -> reinterpret2/1
  reinterpret2/1 -> concatenate/2
  in3/1 -> reinterpret3/1
  reinterpret3/1 -> concatenate/3
  in4/1 -> reinterpret4/1
  reinterpret4/1 -> concatenate/4

== system snap_adc5g_spec_rpi/fft_wideband_real/fft_biplex_real_4x/bi_real_unscr_4x/mirror_spectrum/complex_conj0/munge_in/split ==
  bus_in : Inport
  reinterpret{1..4} (4 alike) : xbsIndex_r4/Reinterpret  force_arith_type=on  arith_type=Unsigned  force_bin_pt=on  bin_pt=0  block_type=reinterpret
  slice1 : xbsIndex_r4/Slice  nbits=18  boolean_output=off  mode=Upper Bit Location + Width  bit1=-54  base1=MSB of Input  bit0=0  base0=LSB of Input  dbl_ovrd=off  block_type=slice
  slice2 : xbsIndex_r4/Slice  nbits=18  boolean_output=off  mode=Upper Bit Location + Width  bit1=-36  base1=MSB of Input  bit0=0  base0=LSB of Input  dbl_ovrd=off  block_type=slice
  slice3 : xbsIndex_r4/Slice  nbits=18  boolean_output=off  mode=Upper Bit Location + Width  bit1=-18  base1=MSB of Input  bit0=0  base0=LSB of Input  dbl_ovrd=off  block_type=slice
  slice4 : xbsIndex_r4/Slice  nbits=18  boolean_output=off  mode=Upper Bit Location + Width  bit1=0  base1=MSB of Input  bit0=0  base0=LSB of Input  dbl_ovrd=off  block_type=slice
  msb_out4 : Outport
  out3 : Outport  Port=2
  out2 : Outport  Port=3
  lsb_out1 : Outport  Port=4
  wires:
  bus_in/1 -> slice4/1, slice3/1, slice2/1, slice1/1
  slice4/1 -> reinterpret4/1
  reinterpret4/1 -> msb_out4/1
  slice3/1 -> reinterpret3/1
  reinterpret3/1 -> out3/1
  slice2/1 -> reinterpret2/1
  reinterpret2/1 -> out2/1
  slice1/1 -> reinterpret1/1
  reinterpret1/1 -> lsb_out1/1

== system snap_adc5g_spec_rpi/fft_wideband_real/fft_biplex_real_4x/bi_real_unscr_4x/mirror_spectrum/complex_conj0/munge_out/join ==
  in1 : Inport
  in2 : Inport  Port=2
  in3 : Inport  Port=3
  in4 : Inport  Port=4
  concatenate : xbsIndex_r4/Concat  num_inputs=4  dbl_ovrd=off  block_type=concat
  reinterpret{1..4} (4 alike) : xbsIndex_r4/Reinterpret  force_arith_type=on  arith_type=Unsigned  force_bin_pt=on  bin_pt=0  block_type=reinterpret
      reinterpret1 settings: infoedit="Changes signal type without altering the binary representation.   You can changed the signal between signed and unsigned, and relocate the binary point.<br><br>Hardware notes: In hardware this block costs nothing.<br><br>Example:  Suppose the input is 6 bits wide, signed, with 2 fractional bits, and the output is forced to unsigned with 0 fractional bits.  Then an input of -2.0 (1110.00 in binary 2's complement) becomes an output of 56 (111000 in binary)."
      reinterpret2 settings: infoedit="Changes signal type without altering the binary representation.   You can changed the signal between signed and unsigned, and relocate the binary point.<br><br>Hardware notes: In hardware this block costs nothing.<br><br>Example:  Suppose the input is 6 bits wide, signed, with 2 fractional bits, and the output is forced to unsigned with 0 fractional bits.  Then an input of -2.0 (1110.00 in binary 2's complement) becomes an output of 56 (111000 in binary)."
  bus_out : Outport
  wires:
  concatenate/1 -> bus_out/1
  in1/1 -> reinterpret1/1
  reinterpret1/1 -> concatenate/1
  in2/1 -> reinterpret2/1
  reinterpret2/1 -> concatenate/2
  in3/1 -> reinterpret3/1
  reinterpret3/1 -> concatenate/3
  in4/1 -> reinterpret4/1
  reinterpret4/1 -> concatenate/4

== system snap_adc5g_spec_rpi/fft_wideband_real/fft_biplex_real_4x/bi_real_unscr_4x/mirror_spectrum/complex_conj0/munge_out/split ==
  bus_in : Inport
  reinterpret{1..4} (4 alike) : xbsIndex_r4/Reinterpret  force_arith_type=on  arith_type=Unsigned  force_bin_pt=on  bin_pt=0  block_type=reinterpret
  slice1 : xbsIndex_r4/Slice  nbits=18  boolean_output=off  mode=Upper Bit Location + Width  bit1=-54  base1=MSB of Input  bit0=0  base0=LSB of Input  dbl_ovrd=off  block_type=slice
  slice2 : xbsIndex_r4/Slice  nbits=18  boolean_output=off  mode=Upper Bit Location + Width  bit1=-36  base1=MSB of Input  bit0=0  base0=LSB of Input  dbl_ovrd=off  block_type=slice
  slice3 : xbsIndex_r4/Slice  nbits=18  boolean_output=off  mode=Upper Bit Location + Width  bit1=-18  base1=MSB of Input  bit0=0  base0=LSB of Input  dbl_ovrd=off  block_type=slice
  slice4 : xbsIndex_r4/Slice  nbits=18  boolean_output=off  mode=Upper Bit Location + Width  bit1=0  base1=MSB of Input  bit0=0  base0=LSB of Input  dbl_ovrd=off  block_type=slice
  msb_out4 : Outport
  out3 : Outport  Port=2
  out2 : Outport  Port=3
  lsb_out1 : Outport  Port=4
  wires:
  bus_in/1 -> slice4/1, slice3/1, slice2/1, slice1/1
  slice4/1 -> reinterpret4/1
  reinterpret4/1 -> msb_out4/1
  slice3/1 -> reinterpret3/1
  reinterpret3/1 -> out3/1
  slice2/1 -> reinterpret2/1
  reinterpret2/1 -> out2/1
  slice1/1 -> reinterpret1/1
  reinterpret1/1 -> lsb_out1/1

== system snap_adc5g_spec_rpi/fft_wideband_real/fft_biplex_real_4x/bi_real_unscr_4x/mirror_spectrum/complex_conj1/imag_negate/bussify ==
  in1 : Inport
  in2 : Inport  Port=2
  concatenate : xbsIndex_r4/Concat  num_inputs=2  dbl_ovrd=off  block_type=concat
  reinterpret1 : xbsIndex_r4/Reinterpret  force_arith_type=on  arith_type=Unsigned  force_bin_pt=on  bin_pt=0  block_type=reinterpret
      settings: infoedit="Changes signal type without altering the binary representation.   You can changed the signal between signed and unsigned, and relocate the binary point.<br><br>Hardware notes: In hardware this block costs nothing.<br><br>Example:  Suppose the input is 6 bits wide, signed, with 2 fractional bits, and the output is forced to unsigned with 0 fractional bits.  Then an input of -2.0 (1110.00 in binary 2's complement) becomes an output of 56 (111000 in binary)."
  reinterpret2 : xbsIndex_r4/Reinterpret  force_arith_type=on  arith_type=Unsigned  force_bin_pt=on  bin_pt=0  block_type=reinterpret
      settings: infoedit="Changes signal type without altering the binary representation.   You can changed the signal between signed and unsigned, and relocate the binary point.<br><br>Hardware notes: In hardware this block costs nothing.<br><br>Example:  Suppose the input is 6 bits wide, signed, with 2 fractional bits, and the output is forced to unsigned with 0 fractional bits.  Then an input of -2.0 (1110.00 in binary 2's complement) becomes an output of 56 (111000 in binary)."
  bus_out : Outport
  wires:
  concatenate/1 -> bus_out/1
  in1/1 -> reinterpret1/1
  reinterpret1/1 -> concatenate/1
  in2/1 -> reinterpret2/1
  reinterpret2/1 -> concatenate/2

== system snap_adc5g_spec_rpi/fft_wideband_real/fft_biplex_real_4x/bi_real_unscr_4x/mirror_spectrum/complex_conj1/imag_negate/debus ==
  bus_in : Inport
  reinterpret1 : xbsIndex_r4/Reinterpret  force_arith_type=on  arith_type="Signed  (2's comp)"  force_bin_pt=on  bin_pt=17  block_type=reinterpret
  reinterpret2 : xbsIndex_r4/Reinterpret  force_arith_type=on  arith_type="Signed  (2's comp)"  force_bin_pt=on  bin_pt=17  block_type=reinterpret
  slice1 : xbsIndex_r4/Slice  nbits=18  boolean_output=off  mode=Upper Bit Location + Width  bit1=-18  base1=MSB of Input  bit0=0  base0=LSB of Input  dbl_ovrd=off  block_type=slice
  slice2 : xbsIndex_r4/Slice  nbits=18  boolean_output=off  mode=Upper Bit Location + Width  bit1=0  base1=MSB of Input  bit0=0  base0=LSB of Input  dbl_ovrd=off  block_type=slice
  msb_out2 : Outport
  lsb_out1 : Outport  Port=2
  wires:
  bus_in/1 -> slice2/1, slice1/1
  slice2/1 -> reinterpret2/1
  reinterpret2/1 -> msb_out2/1
  slice1/1 -> reinterpret1/1
  reinterpret1/1 -> lsb_out1/1

== system snap_adc5g_spec_rpi/fft_wideband_real/fft_biplex_real_4x/bi_real_unscr_4x/mirror_spectrum/complex_conj1/munge_in/join ==
  in1 : Inport
  in2 : Inport  Port=2
  in3 : Inport  Port=3
  in4 : Inport  Port=4
  concatenate : xbsIndex_r4/Concat  num_inputs=4  dbl_ovrd=off  block_type=concat
  reinterpret{1..4} (4 alike) : xbsIndex_r4/Reinterpret  force_arith_type=on  arith_type=Unsigned  force_bin_pt=on  bin_pt=0  block_type=reinterpret
      reinterpret1 settings: infoedit="Changes signal type without altering the binary representation.   You can changed the signal between signed and unsigned, and relocate the binary point.<br><br>Hardware notes: In hardware this block costs nothing.<br><br>Example:  Suppose the input is 6 bits wide, signed, with 2 fractional bits, and the output is forced to unsigned with 0 fractional bits.  Then an input of -2.0 (1110.00 in binary 2's complement) becomes an output of 56 (111000 in binary)."
      reinterpret2 settings: infoedit="Changes signal type without altering the binary representation.   You can changed the signal between signed and unsigned, and relocate the binary point.<br><br>Hardware notes: In hardware this block costs nothing.<br><br>Example:  Suppose the input is 6 bits wide, signed, with 2 fractional bits, and the output is forced to unsigned with 0 fractional bits.  Then an input of -2.0 (1110.00 in binary 2's complement) becomes an output of 56 (111000 in binary)."
  bus_out : Outport
  wires:
  concatenate/1 -> bus_out/1
  in1/1 -> reinterpret1/1
  reinterpret1/1 -> concatenate/1
  in2/1 -> reinterpret2/1
  reinterpret2/1 -> concatenate/2
  in3/1 -> reinterpret3/1
  reinterpret3/1 -> concatenate/3
  in4/1 -> reinterpret4/1
  reinterpret4/1 -> concatenate/4

== system snap_adc5g_spec_rpi/fft_wideband_real/fft_biplex_real_4x/bi_real_unscr_4x/mirror_spectrum/complex_conj1/munge_in/split ==
  bus_in : Inport
  reinterpret{1..4} (4 alike) : xbsIndex_r4/Reinterpret  force_arith_type=on  arith_type=Unsigned  force_bin_pt=on  bin_pt=0  block_type=reinterpret
  slice1 : xbsIndex_r4/Slice  nbits=18  boolean_output=off  mode=Upper Bit Location + Width  bit1=-54  base1=MSB of Input  bit0=0  base0=LSB of Input  dbl_ovrd=off  block_type=slice
  slice2 : xbsIndex_r4/Slice  nbits=18  boolean_output=off  mode=Upper Bit Location + Width  bit1=-36  base1=MSB of Input  bit0=0  base0=LSB of Input  dbl_ovrd=off  block_type=slice
  slice3 : xbsIndex_r4/Slice  nbits=18  boolean_output=off  mode=Upper Bit Location + Width  bit1=-18  base1=MSB of Input  bit0=0  base0=LSB of Input  dbl_ovrd=off  block_type=slice
  slice4 : xbsIndex_r4/Slice  nbits=18  boolean_output=off  mode=Upper Bit Location + Width  bit1=0  base1=MSB of Input  bit0=0  base0=LSB of Input  dbl_ovrd=off  block_type=slice
  msb_out4 : Outport
  out3 : Outport  Port=2
  out2 : Outport  Port=3
  lsb_out1 : Outport  Port=4
  wires:
  bus_in/1 -> slice4/1, slice3/1, slice2/1, slice1/1
  slice4/1 -> reinterpret4/1
  reinterpret4/1 -> msb_out4/1
  slice3/1 -> reinterpret3/1
  reinterpret3/1 -> out3/1
  slice2/1 -> reinterpret2/1
  reinterpret2/1 -> out2/1
  slice1/1 -> reinterpret1/1
  reinterpret1/1 -> lsb_out1/1
